simulink model "rolling_contact_36_example"  (R2026b)
settings: Solver=VariableStepAuto  StopTime=5
undefined symbols (not defined in the file): f_rr, k_gx, k_gy, k_x, m_wheel, miu_p, miu_s, mu_slide, mu_stick, omega_rr_eps, r_wheel, sgn, v_gx_max, v_gy_max, vLimit, X, Y, Z
libraries: nesl_utility x225, sm_lib x156, simulink x146, simulink_extras x36
(part 9 of 11)

== system rolling_contact_36_example/36-Point Sliding Contact Model/Body Contact 18/Ground Friction Model/X-Axis Kinetic Friction Model ==
  note: Sliding Limit Detector
  note: Footpoint Determiner
  note: Kinetic Friction Model
  pos [m] : Inport
  vel [m/s] : Inport  Port=2
  F_Normal [N] : Inport  Port=3
  Enable : EnablePort  StatesWhenEnabling=reset  ZeroCross=off
  Abs : Abs  SaturateOnIntegerOverflow=off
  Constant : Constant  Value=vLimit
  FixPt Relational Operator : RelationalOperator  Operator=>  OutDataTypeStr=boolean  ZeroCross=off  InputSameDT=off
  Memory : Memory
  Negative : simulink/Logic and Bit Operations/Compare To Zero  relop=<  OutDataTypeStr=boolean
  Product : Product  RndMeth=Zero
  Sign1 : Signum
  Sum : Sum  Inputs=|+-
  reverse : Gain  Gain=-1
  sliding friction coefficient : Gain  Gain=mu_slide
  posFP [m] : Outport  InitialOutput=0
      settings: AttributesFormatString=initial = '%<InitialOutput>'\nwhen disabled = '%<OutputWhenDisabled>'
  Stiction! : Outport  Port=2  OutputWhenDisabled=reset  InitialOutput=0
      settings: AttributesFormatString=initial = '%<InitialOutput>'\nwhen disabled = '%<OutputWhenDisabled>'
  F_Slide [N] : Outport  Port=3  OutputWhenDisabled=reset  InitialOutput=0
      settings: AttributesFormatString=initial = '%<InitialOutput>'\nwhen disabled = '%<OutputWhenDisabled>'
  wires:
  Constant/1 -> Sum/2
  Sum/1 -> Negative/1
  Abs/1 -> Sum/1
  Negative/1 -> Memory/1, FixPt Relational Operator/1
  Memory/1 -> FixPt Relational Operator/2
  FixPt Relational Operator/1 -> Stiction!/1
  Sign1/1 -> reverse/1
  sliding friction coefficient/1 -> Product/2
  Product/1 -> F_Slide [N]/1
  pos [m]/1 -> posFP [m]/1
  vel [m/s]/1 -> Abs/1, Sign1/1
  F_Normal [N]/1 -> sliding friction coefficient/1
  reverse/1 -> Product/1

== system rolling_contact_36_example/36-Point Sliding Contact Model/Body Contact 18/Ground Friction Model/X-Axis Static Friction Model ==
  note: Static Friction Model
  note: Stiction Limit Detector
  note: Zero multiplication prevents
      | horizontal friction model from
      | oscillating between static and kinetic
      | friction when the vertical force is zero but
      | the ground level is not yet reached
      | in the upward motion
  F_Normal [N] : Inport
  pos [m] : Inport  Port=2
  vel [m/s] : Inport  Port=3
  posFP [m] : Inport  Port=4
  Enable : EnablePort  StatesWhenEnabling=reset  ZeroCross=off
  Abs : Abs  SaturateOnIntegerOverflow=off
  Abs. : Abs  SaturateOnIntegerOverflow=off
  Check Vertical Friction : Product  RndMeth=Zero
  FixPt Relational Operator : RelationalOperator  Operator=>  OutDataTypeStr=boolean  ZeroCross=off  InputSameDT=off
  Gain3 : Gain  Gain=k_gx
  Gain4 : Gain  Gain=1/v_gx_max
  Memory : Memory
  Mux1 : Mux  Inputs=2
  Positive : simulink/Logic and Bit Operations/Compare To Zero  relop=>  OutDataTypeStr=boolean
  Positive1 : simulink/Logic and Bit Operations/Compare To Zero  relop=>  OutDataTypeStr=boolean
  Sum : Sum  Inputs=-+
  Sum2 : Sum  Inputs=-+|
  X-Axis Stiction Force : Fcn  Expr=-u(1) * (1+sgn(u(1))*u(2))
  stiction limit force : Gain  Gain=mu_stick
  F_Stick [N] : Outport  OutputWhenDisabled=reset  InitialOutput=0
      settings: AttributesFormatString=when disabled: %<OutputWhenDisabled>\ninitial: %<InitialOutput>
  Sliding! : Outport  Port=2  OutputWhenDisabled=reset  InitialOutput=0
      settings: AttributesFormatString=when disabled: %<OutputWhenDisabled>\ninitial: %<InitialOutput>
  wires:
  F_Normal [N]/1 -> stiction limit force/1, Positive1/1
  Sum2/1 -> Gain3/1  "dx"
  pos [m]/1 -> Sum2/2
  posFP [m]/1 -> Sum2/1
  vel [m/s]/1 -> Gain4/1
  Sum/1 -> Positive/1
  Memory/1 -> FixPt Relational Operator/2
  Positive/1 -> FixPt Relational Operator/1, Memory/1
  Abs./1 -> Sum/2
  Mux1/1 -> X-Axis Stiction Force/1
  Gain3/1 -> Mux1/1
  Gain4/1 -> Mux1/2
  FixPt Relational Operator/1 -> Sliding!/1
  Abs/1 -> Sum/1
  stiction limit force/1 -> Abs/1
  X-Axis Stiction Force/1 -> Check Vertical Friction/1
  Positive1/1 -> Check Vertical Friction/2
  Check Vertical Friction/1 -> F_Stick [N]/1, Abs./1

== system rolling_contact_36_example/36-Point Sliding Contact Model/Body Contact 19/Ground Friction Model/Friction Switch ==
  note: Static/Kinetic Friction Switch
  Slide! : Inport
  Stick! : Inport  Port=2
  Memory : Memory
  S-R Flip-Flop : simulink_extras/Flip Flops/S-R Flip-Flop  initial_condition=1
  Terminator : Terminator
  Stiction : Outport
  wires:
  S-R Flip-Flop/1 -> Memory/1
  S-R Flip-Flop/2 -> Terminator/1
  Stick!/1 -> S-R Flip-Flop/1
  Slide!/1 -> S-R Flip-Flop/2
  Memory/1 -> Stiction/1

== system rolling_contact_36_example/36-Point Sliding Contact Model/Body Contact 19/Ground Friction Model/X-Axis Kinetic Friction Model ==
  note: Kinetic Friction Model
  note: Footpoint Determiner
  note: Sliding Limit Detector
  pos [m] : Inport
  vel [m/s] : Inport  Port=2
  F_Normal [N] : Inport  Port=3
  Enable : EnablePort  StatesWhenEnabling=reset  ZeroCross=off
  Abs : Abs  SaturateOnIntegerOverflow=off
  Constant : Constant  Value=vLimit
  FixPt Relational Operator : RelationalOperator  Operator=>  OutDataTypeStr=boolean  ZeroCross=off  InputSameDT=off
  Memory : Memory
  Negative : simulink/Logic and Bit Operations/Compare To Zero  relop=<  OutDataTypeStr=boolean
  Product : Product  RndMeth=Zero
  Sign1 : Signum
  Sum : Sum  Inputs=|+-
  reverse : Gain  Gain=-1
  sliding friction coefficient : Gain  Gain=mu_slide
  posFP [m] : Outport  InitialOutput=0
      settings: AttributesFormatString=initial = '%<InitialOutput>'\nwhen disabled = '%<OutputWhenDisabled>'
  Stiction! : Outport  Port=2  OutputWhenDisabled=reset  InitialOutput=0
      settings: AttributesFormatString=initial = '%<InitialOutput>'\nwhen disabled = '%<OutputWhenDisabled>'
  F_Slide [N] : Outport  Port=3  OutputWhenDisabled=reset  InitialOutput=0
      settings: AttributesFormatString=initial = '%<InitialOutput>'\nwhen disabled = '%<OutputWhenDisabled>'
  wires:
  reverse/1 -> Product/1
  F_Normal [N]/1 -> sliding friction coefficient/1
  vel [m/s]/1 -> Sign1/1, Abs/1
  pos [m]/1 -> posFP [m]/1
  Product/1 -> F_Slide [N]/1
  sliding friction coefficient/1 -> Product/2
  Sign1/1 -> reverse/1
  FixPt Relational Operator/1 -> Stiction!/1
  Memory/1 -> FixPt Relational Operator/2
  Negative/1 -> FixPt Relational Operator/1, Memory/1
  Abs/1 -> Sum/1
  Sum/1 -> Negative/1
  Constant/1 -> Sum/2

== system rolling_contact_36_example/36-Point Sliding Contact Model/Body Contact 19/Ground Friction Model/X-Axis Static Friction Model ==
  note: Zero multiplication prevents
      | horizontal friction model from
      | oscillating between static and kinetic
      | friction when the vertical force is zero but
      | the ground level is not yet reached
      | in the upward motion
  note: Stiction Limit Detector
  note: Static Friction Model
  F_Normal [N] : Inport
  pos [m] : Inport  Port=2
  vel [m/s] : Inport  Port=3
  posFP [m] : Inport  Port=4
  Enable : EnablePort  StatesWhenEnabling=reset  ZeroCross=off
  Abs : Abs  SaturateOnIntegerOverflow=off
  Abs. : Abs  SaturateOnIntegerOverflow=off
  Check Vertical Friction : Product  RndMeth=Zero
  FixPt Relational Operator : RelationalOperator  Operator=>  OutDataTypeStr=boolean  ZeroCross=off  InputSameDT=off
  Gain3 : Gain  Gain=k_gx
  Gain4 : Gain  Gain=1/v_gx_max
  Memory : Memory
  Mux1 : Mux  Inputs=2
  Positive : simulink/Logic and Bit Operations/Compare To Zero  relop=>  OutDataTypeStr=boolean
  Positive1 : simulink/Logic and Bit Operations/Compare To Zero  relop=>  OutDataTypeStr=boolean
  Sum : Sum  Inputs=-+
  Sum2 : Sum  Inputs=-+|
  X-Axis Stiction Force : Fcn  Expr=-u(1) * (1+sgn(u(1))*u(2))
  stiction limit force : Gain  Gain=mu_stick
  F_Stick [N] : Outport  OutputWhenDisabled=reset  InitialOutput=0
      settings: AttributesFormatString=when disabled: %<OutputWhenDisabled>\ninitial: %<InitialOutput>
  Sliding! : Outport  Port=2  OutputWhenDisabled=reset  InitialOutput=0
      settings: AttributesFormatString=when disabled: %<OutputWhenDisabled>\ninitial: %<InitialOutput>
  wires:
  Check Vertical Friction/1 -> Abs./1, F_Stick [N]/1
  Positive1/1 -> Check Vertical Friction/2
  X-Axis Stiction Force/1 -> Check Vertical Friction/1
  stiction limit force/1 -> Abs/1
  Abs/1 -> Sum/1
  FixPt Relational Operator/1 -> Sliding!/1
  Gain4/1 -> Mux1/2
  Gain3/1 -> Mux1/1
  Mux1/1 -> X-Axis Stiction Force/1
  Abs./1 -> Sum/2
  Positive/1 -> Memory/1, FixPt Relational Operator/1
  Memory/1 -> FixPt Relational Operator/2
  Sum/1 -> Positive/1
  vel [m/s]/1 -> Gain4/1
  posFP [m]/1 -> Sum2/1
  pos [m]/1 -> Sum2/2
  Sum2/1 -> Gain3/1  "dx"
  F_Normal [N]/1 -> Positive1/1, stiction limit force/1

== system rolling_contact_36_example/36-Point Sliding Contact Model/Body Contact 2/Ground Friction Model/Friction Switch ==
  note: Static/Kinetic Friction Switch
  Slide! : Inport
  Stick! : Inport  Port=2
  Memory : Memory
  S-R Flip-Flop : simulink_extras/Flip Flops/S-R Flip-Flop  initial_condition=1
  Terminator : Terminator
  Stiction : Outport
  wires:
  Memory/1 -> Stiction/1
  Slide!/1 -> S-R Flip-Flop/2
  Stick!/1 -> S-R Flip-Flop/1
  S-R Flip-Flop/2 -> Terminator/1
  S-R Flip-Flop/1 -> Memory/1

== system rolling_contact_36_example/36-Point Sliding Contact Model/Body Contact 2/Ground Friction Model/X-Axis Kinetic Friction Model ==
  note: Sliding Limit Detector
  note: Footpoint Determiner
  note: Kinetic Friction Model
  pos [m] : Inport
  vel [m/s] : Inport  Port=2
  F_Normal [N] : Inport  Port=3
  Enable : EnablePort  StatesWhenEnabling=reset  ZeroCross=off
  Abs : Abs  SaturateOnIntegerOverflow=off
  Constant : Constant  Value=vLimit
  FixPt Relational Operator : RelationalOperator  Operator=>  OutDataTypeStr=boolean  ZeroCross=off  InputSameDT=off
  Memory : Memory
  Negative : simulink/Logic and Bit Operations/Compare To Zero  relop=<  OutDataTypeStr=boolean
  Product : Product  RndMeth=Zero
  Sign1 : Signum
  Sum : Sum  Inputs=|+-
  reverse : Gain  Gain=-1
  sliding friction coefficient : Gain  Gain=mu_slide
  posFP [m] : Outport  InitialOutput=0
      settings: AttributesFormatString=initial = '%<InitialOutput>'\nwhen disabled = '%<OutputWhenDisabled>'
  Stiction! : Outport  Port=2  OutputWhenDisabled=reset  InitialOutput=0
      settings: AttributesFormatString=initial = '%<InitialOutput>'\nwhen disabled = '%<OutputWhenDisabled>'
  F_Slide [N] : Outport  Port=3  OutputWhenDisabled=reset  InitialOutput=0
      settings: AttributesFormatString=initial = '%<InitialOutput>'\nwhen disabled = '%<OutputWhenDisabled>'
  wires:
  Constant/1 -> Sum/2
  Sum/1 -> Negative/1
  Abs/1 -> Sum/1
  Negative/1 -> Memory/1, FixPt Relational Operator/1
  Memory/1 -> FixPt Relational Operator/2
  FixPt Relational Operator/1 -> Stiction!/1
  Sign1/1 -> reverse/1
  sliding friction coefficient/1 -> Product/2
  Product/1 -> F_Slide [N]/1
  pos [m]/1 -> posFP [m]/1
  vel [m/s]/1 -> Abs/1, Sign1/1
  F_Normal [N]/1 -> sliding friction coefficient/1
  reverse/1 -> Product/1

== system rolling_contact_36_example/36-Point Sliding Contact Model/Body Contact 2/Ground Friction Model/X-Axis Static Friction Model ==
  note: Static Friction Model
  note: Stiction Limit Detector
  note: Zero multiplication prevents
      | horizontal friction model from
      | oscillating between static and kinetic
      | friction when the vertical force is zero but
      | the ground level is not yet reached
      | in the upward motion
  F_Normal [N] : Inport
  pos [m] : Inport  Port=2
  vel [m/s] : Inport  Port=3
  posFP [m] : Inport  Port=4
  Enable : EnablePort  StatesWhenEnabling=reset  ZeroCross=off
  Abs : Abs  SaturateOnIntegerOverflow=off
  Abs. : Abs  SaturateOnIntegerOverflow=off
  Check Vertical Friction : Product  RndMeth=Zero
  FixPt Relational Operator : RelationalOperator  Operator=>  OutDataTypeStr=boolean  ZeroCross=off  InputSameDT=off
  Gain3 : Gain  Gain=k_gx
  Gain4 : Gain  Gain=1/v_gx_max
  Memory : Memory
  Mux1 : Mux  Inputs=2
  Positive : simulink/Logic and Bit Operations/Compare To Zero  relop=>  OutDataTypeStr=boolean
  Positive1 : simulink/Logic and Bit Operations/Compare To Zero  relop=>  OutDataTypeStr=boolean
  Sum : Sum  Inputs=-+
  Sum2 : Sum  Inputs=-+|
  X-Axis Stiction Force : Fcn  Expr=-u(1) * (1+sgn(u(1))*u(2))
  stiction limit force : Gain  Gain=mu_stick
  F_Stick [N] : Outport  OutputWhenDisabled=reset  InitialOutput=0
      settings: AttributesFormatString=when disabled: %<OutputWhenDisabled>\ninitial: %<InitialOutput>
  Sliding! : Outport  Port=2  OutputWhenDisabled=reset  InitialOutput=0
      settings: AttributesFormatString=when disabled: %<OutputWhenDisabled>\ninitial: %<InitialOutput>
  wires:
  F_Normal [N]/1 -> stiction limit force/1, Positive1/1
  Sum2/1 -> Gain3/1  "dx"
  pos [m]/1 -> Sum2/2
  posFP [m]/1 -> Sum2/1
  vel [m/s]/1 -> Gain4/1
  Sum/1 -> Positive/1
  Memory/1 -> FixPt Relational Operator/2
  Positive/1 -> FixPt Relational Operator/1, Memory/1
  Abs./1 -> Sum/2
  Mux1/1 -> X-Axis Stiction Force/1
  Gain3/1 -> Mux1/1
  Gain4/1 -> Mux1/2
  FixPt Relational Operator/1 -> Sliding!/1
  Abs/1 -> Sum/1
  stiction limit force/1 -> Abs/1
  X-Axis Stiction Force/1 -> Check Vertical Friction/1
  Positive1/1 -> Check Vertical Friction/2
  Check Vertical Friction/1 -> F_Stick [N]/1, Abs./1

== system rolling_contact_36_example/36-Point Sliding Contact Model/Body Contact 20/Ground Friction Model/Friction Switch ==
  note: Static/Kinetic Friction Switch
  Slide! : Inport
  Stick! : Inport  Port=2
  Memory : Memory
  S-R Flip-Flop : simulink_extras/Flip Flops/S-R Flip-Flop  initial_condition=1
  Terminator : Terminator
  Stiction : Outport
  wires:
  Memory/1 -> Stiction/1
  Slide!/1 -> S-R Flip-Flop/2
  Stick!/1 -> S-R Flip-Flop/1
  S-R Flip-Flop/2 -> Terminator/1
  S-R Flip-Flop/1 -> Memory/1

== system rolling_contact_36_example/36-Point Sliding Contact Model/Body Contact 20/Ground Friction Model/X-Axis Kinetic Friction Model ==
  note: Sliding Limit Detector
  note: Footpoint Determiner
  note: Kinetic Friction Model
  pos [m] : Inport
  vel [m/s] : Inport  Port=2
  F_Normal [N] : Inport  Port=3
  Enable : EnablePort  StatesWhenEnabling=reset  ZeroCross=off
  Abs : Abs  SaturateOnIntegerOverflow=off
  Constant : Constant  Value=vLimit
  FixPt Relational Operator : RelationalOperator  Operator=>  OutDataTypeStr=boolean  ZeroCross=off  InputSameDT=off
  Memory : Memory
  Negative : simulink/Logic and Bit Operations/Compare To Zero  relop=<  OutDataTypeStr=boolean
  Product : Product  RndMeth=Zero
  Sign1 : Signum
  Sum : Sum  Inputs=|+-
  reverse : Gain  Gain=-1
  sliding friction coefficient : Gain  Gain=mu_slide
  posFP [m] : Outport  InitialOutput=0
      settings: AttributesFormatString=initial = '%<InitialOutput>'\nwhen disabled = '%<OutputWhenDisabled>'
  Stiction! : Outport  Port=2  OutputWhenDisabled=reset  InitialOutput=0
      settings: AttributesFormatString=initial = '%<InitialOutput>'\nwhen disabled = '%<OutputWhenDisabled>'
  F_Slide [N] : Outport  Port=3  OutputWhenDisabled=reset  InitialOutput=0
      settings: AttributesFormatString=initial = '%<InitialOutput>'\nwhen disabled = '%<OutputWhenDisabled>'
  wires:
  Constant/1 -> Sum/2
  Sum/1 -> Negative/1
  Abs/1 -> Sum/1
  Negative/1 -> Memory/1, FixPt Relational Operator/1
  Memory/1 -> FixPt Relational Operator/2
  FixPt Relational Operator/1 -> Stiction!/1
  Sign1/1 -> reverse/1
  sliding friction coefficient/1 -> Product/2
  Product/1 -> F_Slide [N]/1
  pos [m]/1 -> posFP [m]/1
  vel [m/s]/1 -> Abs/1, Sign1/1
  F_Normal [N]/1 -> sliding friction coefficient/1
  reverse/1 -> Product/1

== system rolling_contact_36_example/36-Point Sliding Contact Model/Body Contact 20/Ground Friction Model/X-Axis Static Friction Model ==
  note: Static Friction Model
  note: Stiction Limit Detector
  note: Zero multiplication prevents
      | horizontal friction model from
      | oscillating between static and kinetic
      | friction when the vertical force is zero but
      | the ground level is not yet reached
      | in the upward motion
  F_Normal [N] : Inport
  pos [m] : Inport  Port=2
  vel [m/s] : Inport  Port=3
  posFP [m] : Inport  Port=4
  Enable : EnablePort  StatesWhenEnabling=reset  ZeroCross=off
  Abs : Abs  SaturateOnIntegerOverflow=off
  Abs. : Abs  SaturateOnIntegerOverflow=off
  Check Vertical Friction : Product  RndMeth=Zero
  FixPt Relational Operator : RelationalOperator  Operator=>  OutDataTypeStr=boolean  ZeroCross=off  InputSameDT=off
  Gain3 : Gain  Gain=k_gx
  Gain4 : Gain  Gain=1/v_gx_max
  Memory : Memory
  Mux1 : Mux  Inputs=2
  Positive : simulink/Logic and Bit Operations/Compare To Zero  relop=>  OutDataTypeStr=boolean
  Positive1 : simulink/Logic and Bit Operations/Compare To Zero  relop=>  OutDataTypeStr=boolean
  Sum : Sum  Inputs=-+
  Sum2 : Sum  Inputs=-+|
  X-Axis Stiction Force : Fcn  Expr=-u(1) * (1+sgn(u(1))*u(2))
  stiction limit force : Gain  Gain=mu_stick
  F_Stick [N] : Outport  OutputWhenDisabled=reset  InitialOutput=0
      settings: AttributesFormatString=when disabled: %<OutputWhenDisabled>\ninitial: %<InitialOutput>
  Sliding! : Outport  Port=2  OutputWhenDisabled=reset  InitialOutput=0
      settings: AttributesFormatString=when disabled: %<OutputWhenDisabled>\ninitial: %<InitialOutput>
  wires:
  F_Normal [N]/1 -> stiction limit force/1, Positive1/1
  Sum2/1 -> Gain3/1  "dx"
  pos [m]/1 -> Sum2/2
  posFP [m]/1 -> Sum2/1
  vel [m/s]/1 -> Gain4/1
  Sum/1 -> Positive/1
  Memory/1 -> FixPt Relational Operator/2
  Positive/1 -> FixPt Relational Operator/1, Memory/1
  Abs./1 -> Sum/2
  Mux1/1 -> X-Axis Stiction Force/1
  Gain3/1 -> Mux1/1
  Gain4/1 -> Mux1/2
  FixPt Relational Operator/1 -> Sliding!/1
  Abs/1 -> Sum/1
  stiction limit force/1 -> Abs/1
  X-Axis Stiction Force/1 -> Check Vertical Friction/1
  Positive1/1 -> Check Vertical Friction/2
  Check Vertical Friction/1 -> F_Stick [N]/1, Abs./1

== system rolling_contact_36_example/36-Point Sliding Contact Model/Body Contact 21/Ground Friction Model/Friction Switch ==
  note: Static/Kinetic Friction Switch
  Slide! : Inport
  Stick! : Inport  Port=2
  Memory : Memory
  S-R Flip-Flop : simulink_extras/Flip Flops/S-R Flip-Flop  initial_condition=1
  Terminator : Terminator
  Stiction : Outport
  wires:
  S-R Flip-Flop/1 -> Memory/1
  S-R Flip-Flop/2 -> Terminator/1
  Stick!/1 -> S-R Flip-Flop/1
  Slide!/1 -> S-R Flip-Flop/2
  Memory/1 -> Stiction/1

== system rolling_contact_36_example/36-Point Sliding Contact Model/Body Contact 21/Ground Friction Model/X-Axis Kinetic Friction Model ==
  note: Kinetic Friction Model
  note: Footpoint Determiner
  note: Sliding Limit Detector
  pos [m] : Inport
  vel [m/s] : Inport  Port=2
  F_Normal [N] : Inport  Port=3
  Enable : EnablePort  StatesWhenEnabling=reset  ZeroCross=off
  Abs : Abs  SaturateOnIntegerOverflow=off
  Constant : Constant  Value=vLimit
  FixPt Relational Operator : RelationalOperator  Operator=>  OutDataTypeStr=boolean  ZeroCross=off  InputSameDT=off
  Memory : Memory
  Negative : simulink/Logic and Bit Operations/Compare To Zero  relop=<  OutDataTypeStr=boolean
  Product : Product  RndMeth=Zero
  Sign1 : Signum
  Sum : Sum  Inputs=|+-
  reverse : Gain  Gain=-1
  sliding friction coefficient : Gain  Gain=mu_slide
  posFP [m] : Outport  InitialOutput=0
      settings: AttributesFormatString=initial = '%<InitialOutput>'\nwhen disabled = '%<OutputWhenDisabled>'
  Stiction! : Outport  Port=2  OutputWhenDisabled=reset  InitialOutput=0
      settings: AttributesFormatString=initial = '%<InitialOutput>'\nwhen disabled = '%<OutputWhenDisabled>'
  F_Slide [N] : Outport  Port=3  OutputWhenDisabled=reset  InitialOutput=0
      settings: AttributesFormatString=initial = '%<InitialOutput>'\nwhen disabled = '%<OutputWhenDisabled>'
  wires:
  reverse/1 -> Product/1
  F_Normal [N]/1 -> sliding friction coefficient/1
  vel [m/s]/1 -> Sign1/1, Abs/1
  pos [m]/1 -> posFP [m]/1
  Product/1 -> F_Slide [N]/1
  sliding friction coefficient/1 -> Product/2
  Sign1/1 -> reverse/1
  FixPt Relational Operator/1 -> Stiction!/1
  Memory/1 -> FixPt Relational Operator/2
  Negative/1 -> FixPt Relational Operator/1, Memory/1
  Abs/1 -> Sum/1
  Sum/1 -> Negative/1
  Constant/1 -> Sum/2

== system rolling_contact_36_example/36-Point Sliding Contact Model/Body Contact 21/Ground Friction Model/X-Axis Static Friction Model ==
  note: Zero multiplication prevents
      | horizontal friction model from
      | oscillating between static and kinetic
      | friction when the vertical force is zero but
      | the ground level is not yet reached
      | in the upward motion
  note: Stiction Limit Detector
  note: Static Friction Model
  F_Normal [N] : Inport
  pos [m] : Inport  Port=2
  vel [m/s] : Inport  Port=3
  posFP [m] : Inport  Port=4
  Enable : EnablePort  StatesWhenEnabling=reset  ZeroCross=off
  Abs : Abs  SaturateOnIntegerOverflow=off
  Abs. : Abs  SaturateOnIntegerOverflow=off
  Check Vertical Friction : Product  RndMeth=Zero
  FixPt Relational Operator : RelationalOperator  Operator=>  OutDataTypeStr=boolean  ZeroCross=off  InputSameDT=off
  Gain3 : Gain  Gain=k_gx
  Gain4 : Gain  Gain=1/v_gx_max
  Memory : Memory
  Mux1 : Mux  Inputs=2
  Positive : simulink/Logic and Bit Operations/Compare To Zero  relop=>  OutDataTypeStr=boolean
  Positive1 : simulink/Logic and Bit Operations/Compare To Zero  relop=>  OutDataTypeStr=boolean
  Sum : Sum  Inputs=-+
  Sum2 : Sum  Inputs=-+|
  X-Axis Stiction Force : Fcn  Expr=-u(1) * (1+sgn(u(1))*u(2))
  stiction limit force : Gain  Gain=mu_stick
  F_Stick [N] : Outport  OutputWhenDisabled=reset  InitialOutput=0
      settings: AttributesFormatString=when disabled: %<OutputWhenDisabled>\ninitial: %<InitialOutput>
  Sliding! : Outport  Port=2  OutputWhenDisabled=reset  InitialOutput=0
      settings: AttributesFormatString=when disabled: %<OutputWhenDisabled>\ninitial: %<InitialOutput>
  wires:
  Check Vertical Friction/1 -> Abs./1, F_Stick [N]/1
  Positive1/1 -> Check Vertical Friction/2
  X-Axis Stiction Force/1 -> Check Vertical Friction/1
  stiction limit force/1 -> Abs/1
  Abs/1 -> Sum/1
  FixPt Relational Operator/1 -> Sliding!/1
  Gain4/1 -> Mux1/2
  Gain3/1 -> Mux1/1
  Mux1/1 -> X-Axis Stiction Force/1
  Abs./1 -> Sum/2
  Positive/1 -> Memory/1, FixPt Relational Operator/1
  Memory/1 -> FixPt Relational Operator/2
  Sum/1 -> Positive/1
  vel [m/s]/1 -> Gain4/1
  posFP [m]/1 -> Sum2/1
  pos [m]/1 -> Sum2/2
  Sum2/1 -> Gain3/1  "dx"
  F_Normal [N]/1 -> Positive1/1, stiction limit force/1

== system rolling_contact_36_example/36-Point Sliding Contact Model/Body Contact 22/Ground Friction Model/Friction Switch ==
  note: Static/Kinetic Friction Switch
  Slide! : Inport
  Stick! : Inport  Port=2
  Memory : Memory
  S-R Flip-Flop : simulink_extras/Flip Flops/S-R Flip-Flop  initial_condition=1
  Terminator : Terminator
  Stiction : Outport
  wires:
  Memory/1 -> Stiction/1
  Slide!/1 -> S-R Flip-Flop/2
  Stick!/1 -> S-R Flip-Flop/1
  S-R Flip-Flop/2 -> Terminator/1
  S-R Flip-Flop/1 -> Memory/1

== system rolling_contact_36_example/36-Point Sliding Contact Model/Body Contact 22/Ground Friction Model/X-Axis Kinetic Friction Model ==
  note: Sliding Limit Detector
  note: Footpoint Determiner
  note: Kinetic Friction Model
  pos [m] : Inport
  vel [m/s] : Inport  Port=2
  F_Normal [N] : Inport  Port=3
  Enable : EnablePort  StatesWhenEnabling=reset  ZeroCross=off
  Abs : Abs  SaturateOnIntegerOverflow=off
  Constant : Constant  Value=vLimit
  FixPt Relational Operator : RelationalOperator  Operator=>  OutDataTypeStr=boolean  ZeroCross=off  InputSameDT=off
  Memory : Memory
  Negative : simulink/Logic and Bit Operations/Compare To Zero  relop=<  OutDataTypeStr=boolean
  Product : Product  RndMeth=Zero
  Sign1 : Signum
  Sum : Sum  Inputs=|+-
  reverse : Gain  Gain=-1
  sliding friction coefficient : Gain  Gain=mu_slide
  posFP [m] : Outport  InitialOutput=0
      settings: AttributesFormatString=initial = '%<InitialOutput>'\nwhen disabled = '%<OutputWhenDisabled>'
  Stiction! : Outport  Port=2  OutputWhenDisabled=reset  InitialOutput=0
      settings: AttributesFormatString=initial = '%<InitialOutput>'\nwhen disabled = '%<OutputWhenDisabled>'
  F_Slide [N] : Outport  Port=3  OutputWhenDisabled=reset  InitialOutput=0
      settings: AttributesFormatString=initial = '%<InitialOutput>'\nwhen disabled = '%<OutputWhenDisabled>'
  wires:
  Constant/1 -> Sum/2
  Sum/1 -> Negative/1
  Abs/1 -> Sum/1
  Negative/1 -> Memory/1, FixPt Relational Operator/1
  Memory/1 -> FixPt Relational Operator/2
  FixPt Relational Operator/1 -> Stiction!/1
  Sign1/1 -> reverse/1
  sliding friction coefficient/1 -> Product/2
  Product/1 -> F_Slide [N]/1
  pos [m]/1 -> posFP [m]/1
  vel [m/s]/1 -> Abs/1, Sign1/1
  F_Normal [N]/1 -> sliding friction coefficient/1
  reverse/1 -> Product/1

== system rolling_contact_36_example/36-Point Sliding Contact Model/Body Contact 22/Ground Friction Model/X-Axis Static Friction Model ==
  note: Static Friction Model
  note: Stiction Limit Detector
  note: Zero multiplication prevents
      | horizontal friction model from
      | oscillating between static and kinetic
      | friction when the vertical force is zero but
      | the ground level is not yet reached
      | in the upward motion
  F_Normal [N] : Inport
  pos [m] : Inport  Port=2
  vel [m/s] : Inport  Port=3
  posFP [m] : Inport  Port=4
  Enable : EnablePort  StatesWhenEnabling=reset  ZeroCross=off
  Abs : Abs  SaturateOnIntegerOverflow=off
  Abs. : Abs  SaturateOnIntegerOverflow=off
  Check Vertical Friction : Product  RndMeth=Zero
  FixPt Relational Operator : RelationalOperator  Operator=>  OutDataTypeStr=boolean  ZeroCross=off  InputSameDT=off
  Gain3 : Gain  Gain=k_gx
  Gain4 : Gain  Gain=1/v_gx_max
  Memory : Memory
  Mux1 : Mux  Inputs=2
  Positive : simulink/Logic and Bit Operations/Compare To Zero  relop=>  OutDataTypeStr=boolean
  Positive1 : simulink/Logic and Bit Operations/Compare To Zero  relop=>  OutDataTypeStr=boolean
  Sum : Sum  Inputs=-+
  Sum2 : Sum  Inputs=-+|
  X-Axis Stiction Force : Fcn  Expr=-u(1) * (1+sgn(u(1))*u(2))
  stiction limit force : Gain  Gain=mu_stick
  F_Stick [N] : Outport  OutputWhenDisabled=reset  InitialOutput=0
      settings: AttributesFormatString=when disabled: %<OutputWhenDisabled>\ninitial: %<InitialOutput>
  Sliding! : Outport  Port=2  OutputWhenDisabled=reset  InitialOutput=0
      settings: AttributesFormatString=when disabled: %<OutputWhenDisabled>\ninitial: %<InitialOutput>
  wires:
  F_Normal [N]/1 -> stiction limit force/1, Positive1/1
  Sum2/1 -> Gain3/1  "dx"
  pos [m]/1 -> Sum2/2
  posFP [m]/1 -> Sum2/1
  vel [m/s]/1 -> Gain4/1
  Sum/1 -> Positive/1
  Memory/1 -> FixPt Relational Operator/2
  Positive/1 -> FixPt Relational Operator/1, Memory/1
  Abs./1 -> Sum/2
  Mux1/1 -> X-Axis Stiction Force/1
  Gain3/1 -> Mux1/1
  Gain4/1 -> Mux1/2
  FixPt Relational Operator/1 -> Sliding!/1
  Abs/1 -> Sum/1
  stiction limit force/1 -> Abs/1
  X-Axis Stiction Force/1 -> Check Vertical Friction/1
  Positive1/1 -> Check Vertical Friction/2
  Check Vertical Friction/1 -> F_Stick [N]/1, Abs./1

== system rolling_contact_36_example/36-Point Sliding Contact Model/Body Contact 23/Ground Friction Model/Friction Switch ==
  note: Static/Kinetic Friction Switch
  Slide! : Inport
  Stick! : Inport  Port=2
  Memory : Memory
  S-R Flip-Flop : simulink_extras/Flip Flops/S-R Flip-Flop  initial_condition=1
  Terminator : Terminator
  Stiction : Outport
  wires:
  S-R Flip-Flop/1 -> Memory/1
  S-R Flip-Flop/2 -> Terminator/1
  Stick!/1 -> S-R Flip-Flop/1
  Slide!/1 -> S-R Flip-Flop/2
  Memory/1 -> Stiction/1

== system rolling_contact_36_example/36-Point Sliding Contact Model/Body Contact 23/Ground Friction Model/X-Axis Kinetic Friction Model ==
  note: Kinetic Friction Model
  note: Footpoint Determiner
  note: Sliding Limit Detector
  pos [m] : Inport
  vel [m/s] : Inport  Port=2
  F_Normal [N] : Inport  Port=3
  Enable : EnablePort  StatesWhenEnabling=reset  ZeroCross=off
  Abs : Abs  SaturateOnIntegerOverflow=off
  Constant : Constant  Value=vLimit
  FixPt Relational Operator : RelationalOperator  Operator=>  OutDataTypeStr=boolean  ZeroCross=off  InputSameDT=off
  Memory : Memory
  Negative : simulink/Logic and Bit Operations/Compare To Zero  relop=<  OutDataTypeStr=boolean
  Product : Product  RndMeth=Zero
  Sign1 : Signum
  Sum : Sum  Inputs=|+-
  reverse : Gain  Gain=-1
  sliding friction coefficient : Gain  Gain=mu_slide
  posFP [m] : Outport  InitialOutput=0
      settings: AttributesFormatString=initial = '%<InitialOutput>'\nwhen disabled = '%<OutputWhenDisabled>'
  Stiction! : Outport  Port=2  OutputWhenDisabled=reset  InitialOutput=0
      settings: AttributesFormatString=initial = '%<InitialOutput>'\nwhen disabled = '%<OutputWhenDisabled>'
  F_Slide [N] : Outport  Port=3  OutputWhenDisabled=reset  InitialOutput=0
      settings: AttributesFormatString=initial = '%<InitialOutput>'\nwhen disabled = '%<OutputWhenDisabled>'
  wires:
  reverse/1 -> Product/1
  F_Normal [N]/1 -> sliding friction coefficient/1
  vel [m/s]/1 -> Sign1/1, Abs/1
  pos [m]/1 -> posFP [m]/1
  Product/1 -> F_Slide [N]/1
  sliding friction coefficient/1 -> Product/2
  Sign1/1 -> reverse/1
  FixPt Relational Operator/1 -> Stiction!/1
  Memory/1 -> FixPt Relational Operator/2
  Negative/1 -> FixPt Relational Operator/1, Memory/1
  Abs/1 -> Sum/1
  Sum/1 -> Negative/1
  Constant/1 -> Sum/2

== system rolling_contact_36_example/36-Point Sliding Contact Model/Body Contact 23/Ground Friction Model/X-Axis Static Friction Model ==
  note: Zero multiplication prevents
      | horizontal friction model from
      | oscillating between static and kinetic
      | friction when the vertical force is zero but
      | the ground level is not yet reached
      | in the upward motion
  note: Stiction Limit Detector
  note: Static Friction Model
  F_Normal [N] : Inport
  pos [m] : Inport  Port=2
  vel [m/s] : Inport  Port=3
  posFP [m] : Inport  Port=4
  Enable : EnablePort  StatesWhenEnabling=reset  ZeroCross=off
  Abs : Abs  SaturateOnIntegerOverflow=off
  Abs. : Abs  SaturateOnIntegerOverflow=off
  Check Vertical Friction : Product  RndMeth=Zero
  FixPt Relational Operator : RelationalOperator  Operator=>  OutDataTypeStr=boolean  ZeroCross=off  InputSameDT=off
  Gain3 : Gain  Gain=k_gx
  Gain4 : Gain  Gain=1/v_gx_max
  Memory : Memory
  Mux1 : Mux  Inputs=2
  Positive : simulink/Logic and Bit Operations/Compare To Zero  relop=>  OutDataTypeStr=boolean
  Positive1 : simulink/Logic and Bit Operations/Compare To Zero  relop=>  OutDataTypeStr=boolean
  Sum : Sum  Inputs=-+
  Sum2 : Sum  Inputs=-+|
  X-Axis Stiction Force : Fcn  Expr=-u(1) * (1+sgn(u(1))*u(2))
  stiction limit force : Gain  Gain=mu_stick
  F_Stick [N] : Outport  OutputWhenDisabled=reset  InitialOutput=0
      settings: AttributesFormatString=when disabled: %<OutputWhenDisabled>\ninitial: %<InitialOutput>
  Sliding! : Outport  Port=2  OutputWhenDisabled=reset  InitialOutput=0
      settings: AttributesFormatString=when disabled: %<OutputWhenDisabled>\ninitial: %<InitialOutput>
  wires:
  Check Vertical Friction/1 -> Abs./1, F_Stick [N]/1
  Positive1/1 -> Check Vertical Friction/2
  X-Axis Stiction Force/1 -> Check Vertical Friction/1
  stiction limit force/1 -> Abs/1
  Abs/1 -> Sum/1
  FixPt Relational Operator/1 -> Sliding!/1
  Gain4/1 -> Mux1/2
  Gain3/1 -> Mux1/1
  Mux1/1 -> X-Axis Stiction Force/1
  Abs./1 -> Sum/2
  Positive/1 -> Memory/1, FixPt Relational Operator/1
  Memory/1 -> FixPt Relational Operator/2
  Sum/1 -> Positive/1
  vel [m/s]/1 -> Gain4/1
  posFP [m]/1 -> Sum2/1
  pos [m]/1 -> Sum2/2
  Sum2/1 -> Gain3/1  "dx"
  F_Normal [N]/1 -> Positive1/1, stiction limit force/1

== system rolling_contact_36_example/36-Point Sliding Contact Model/Body Contact 24/Ground Friction Model/Friction Switch ==
  note: Static/Kinetic Friction Switch
  Slide! : Inport
  Stick! : Inport  Port=2
  Memory : Memory
  S-R Flip-Flop : simulink_extras/Flip Flops/S-R Flip-Flop  initial_condition=1
  Terminator : Terminator
  Stiction : Outport
  wires:
  Memory/1 -> Stiction/1
  Slide!/1 -> S-R Flip-Flop/2
  Stick!/1 -> S-R Flip-Flop/1
  S-R Flip-Flop/2 -> Terminator/1
  S-R Flip-Flop/1 -> Memory/1

== system rolling_contact_36_example/36-Point Sliding Contact Model/Body Contact 24/Ground Friction Model/X-Axis Kinetic Friction Model ==
  note: Sliding Limit Detector
  note: Footpoint Determiner
  note: Kinetic Friction Model
  pos [m] : Inport
  vel [m/s] : Inport  Port=2
  F_Normal [N] : Inport  Port=3
  Enable : EnablePort  StatesWhenEnabling=reset  ZeroCross=off
  Abs : Abs  SaturateOnIntegerOverflow=off
  Constant : Constant  Value=vLimit
  FixPt Relational Operator : RelationalOperator  Operator=>  OutDataTypeStr=boolean  ZeroCross=off  InputSameDT=off
  Memory : Memory
  Negative : simulink/Logic and Bit Operations/Compare To Zero  relop=<  OutDataTypeStr=boolean
  Product : Product  RndMeth=Zero
  Sign1 : Signum
  Sum : Sum  Inputs=|+-
  reverse : Gain  Gain=-1
  sliding friction coefficient : Gain  Gain=mu_slide
  posFP [m] : Outport  InitialOutput=0
      settings: AttributesFormatString=initial = '%<InitialOutput>'\nwhen disabled = '%<OutputWhenDisabled>'
  Stiction! : Outport  Port=2  OutputWhenDisabled=reset  InitialOutput=0
      settings: AttributesFormatString=initial = '%<InitialOutput>'\nwhen disabled = '%<OutputWhenDisabled>'
  F_Slide [N] : Outport  Port=3  OutputWhenDisabled=reset  InitialOutput=0
      settings: AttributesFormatString=initial = '%<InitialOutput>'\nwhen disabled = '%<OutputWhenDisabled>'
  wires:
  Constant/1 -> Sum/2
  Sum/1 -> Negative/1
  Abs/1 -> Sum/1
  Negative/1 -> Memory/1, FixPt Relational Operator/1
  Memory/1 -> FixPt Relational Operator/2
  FixPt Relational Operator/1 -> Stiction!/1
  Sign1/1 -> reverse/1
  sliding friction coefficient/1 -> Product/2
  Product/1 -> F_Slide [N]/1
  pos [m]/1 -> posFP [m]/1
  vel [m/s]/1 -> Abs/1, Sign1/1
  F_Normal [N]/1 -> sliding friction coefficient/1
  reverse/1 -> Product/1

== system rolling_contact_36_example/36-Point Sliding Contact Model/Body Contact 24/Ground Friction Model/X-Axis Static Friction Model ==
  note: Static Friction Model
  note: Stiction Limit Detector
  note: Zero multiplication prevents
      | horizontal friction model from
      | oscillating between static and kinetic
      | friction when the vertical force is zero but
      | the ground level is not yet reached
      | in the upward motion
  F_Normal [N] : Inport
  pos [m] : Inport  Port=2
  vel [m/s] : Inport  Port=3
  posFP [m] : Inport  Port=4
  Enable : EnablePort  StatesWhenEnabling=reset  ZeroCross=off
  Abs : Abs  SaturateOnIntegerOverflow=off
  Abs. : Abs  SaturateOnIntegerOverflow=off
  Check Vertical Friction : Product  RndMeth=Zero
  FixPt Relational Operator : RelationalOperator  Operator=>  OutDataTypeStr=boolean  ZeroCross=off  InputSameDT=off
  Gain3 : Gain  Gain=k_gx
  Gain4 : Gain  Gain=1/v_gx_max
  Memory : Memory
  Mux1 : Mux  Inputs=2
  Positive : simulink/Logic and Bit Operations/Compare To Zero  relop=>  OutDataTypeStr=boolean
  Positive1 : simulink/Logic and Bit Operations/Compare To Zero  relop=>  OutDataTypeStr=boolean
  Sum : Sum  Inputs=-+
  Sum2 : Sum  Inputs=-+|
  X-Axis Stiction Force : Fcn  Expr=-u(1) * (1+sgn(u(1))*u(2))
  stiction limit force : Gain  Gain=mu_stick
  F_Stick [N] : Outport  OutputWhenDisabled=reset  InitialOutput=0
      settings: AttributesFormatString=when disabled: %<OutputWhenDisabled>\ninitial: %<InitialOutput>
  Sliding! : Outport  Port=2  OutputWhenDisabled=reset  InitialOutput=0
      settings: AttributesFormatString=when disabled: %<OutputWhenDisabled>\ninitial: %<InitialOutput>
  wires:
  F_Normal [N]/1 -> stiction limit force/1, Positive1/1
  Sum2/1 -> Gain3/1  "dx"
  pos [m]/1 -> Sum2/2
  posFP [m]/1 -> Sum2/1
  vel [m/s]/1 -> Gain4/1
  Sum/1 -> Positive/1
  Memory/1 -> FixPt Relational Operator/2
  Positive/1 -> FixPt Relational Operator/1, Memory/1
  Abs./1 -> Sum/2
  Mux1/1 -> X-Axis Stiction Force/1
  Gain3/1 -> Mux1/1
  Gain4/1 -> Mux1/2
  FixPt Relational Operator/1 -> Sliding!/1
  Abs/1 -> Sum/1
  stiction limit force/1 -> Abs/1
  X-Axis Stiction Force/1 -> Check Vertical Friction/1
  Positive1/1 -> Check Vertical Friction/2
  Check Vertical Friction/1 -> F_Stick [N]/1, Abs./1

== system rolling_contact_36_example/36-Point Sliding Contact Model/Body Contact 25/Ground Friction Model/Friction Switch ==
  note: Static/Kinetic Friction Switch
  Slide! : Inport
  Stick! : Inport  Port=2
  Memory : Memory
  S-R Flip-Flop : simulink_extras/Flip Flops/S-R Flip-Flop  initial_condition=1
  Terminator : Terminator
  Stiction : Outport
  wires:
  S-R Flip-Flop/1 -> Memory/1
  S-R Flip-Flop/2 -> Terminator/1
  Stick!/1 -> S-R Flip-Flop/1
  Slide!/1 -> S-R Flip-Flop/2
  Memory/1 -> Stiction/1

== system rolling_contact_36_example/36-Point Sliding Contact Model/Body Contact 25/Ground Friction Model/X-Axis Kinetic Friction Model ==
  note: Kinetic Friction Model
  note: Footpoint Determiner
  note: Sliding Limit Detector
  pos [m] : Inport
  vel [m/s] : Inport  Port=2
  F_Normal [N] : Inport  Port=3
  Enable : EnablePort  StatesWhenEnabling=reset  ZeroCross=off
  Abs : Abs  SaturateOnIntegerOverflow=off
  Constant : Constant  Value=vLimit
  FixPt Relational Operator : RelationalOperator  Operator=>  OutDataTypeStr=boolean  ZeroCross=off  InputSameDT=off
  Memory : Memory
  Negative : simulink/Logic and Bit Operations/Compare To Zero  relop=<  OutDataTypeStr=boolean
  Product : Product  RndMeth=Zero
  Sign1 : Signum
  Sum : Sum  Inputs=|+-
  reverse : Gain  Gain=-1
  sliding friction coefficient : Gain  Gain=mu_slide
  posFP [m] : Outport  InitialOutput=0
      settings: AttributesFormatString=initial = '%<InitialOutput>'\nwhen disabled = '%<OutputWhenDisabled>'
  Stiction! : Outport  Port=2  OutputWhenDisabled=reset  InitialOutput=0
      settings: AttributesFormatString=initial = '%<InitialOutput>'\nwhen disabled = '%<OutputWhenDisabled>'
  F_Slide [N] : Outport  Port=3  OutputWhenDisabled=reset  InitialOutput=0
      settings: AttributesFormatString=initial = '%<InitialOutput>'\nwhen disabled = '%<OutputWhenDisabled>'
  wires:
  reverse/1 -> Product/1
  F_Normal [N]/1 -> sliding friction coefficient/1
  vel [m/s]/1 -> Sign1/1, Abs/1
  pos [m]/1 -> posFP [m]/1
  Product/1 -> F_Slide [N]/1
  sliding friction coefficient/1 -> Product/2
  Sign1/1 -> reverse/1
  FixPt Relational Operator/1 -> Stiction!/1
  Memory/1 -> FixPt Relational Operator/2
  Negative/1 -> FixPt Relational Operator/1, Memory/1
  Abs/1 -> Sum/1
  Sum/1 -> Negative/1
  Constant/1 -> Sum/2

== system rolling_contact_36_example/36-Point Sliding Contact Model/Body Contact 25/Ground Friction Model/X-Axis Static Friction Model ==
  note: Zero multiplication prevents
      | horizontal friction model from
      | oscillating between static and kinetic
      | friction when the vertical force is zero but
      | the ground level is not yet reached
      | in the upward motion
  note: Stiction Limit Detector
  note: Static Friction Model
  F_Normal [N] : Inport
  pos [m] : Inport  Port=2
  vel [m/s] : Inport  Port=3
  posFP [m] : Inport  Port=4
  Enable : EnablePort  StatesWhenEnabling=reset  ZeroCross=off
  Abs : Abs  SaturateOnIntegerOverflow=off
  Abs. : Abs  SaturateOnIntegerOverflow=off
  Check Vertical Friction : Product  RndMeth=Zero
  FixPt Relational Operator : RelationalOperator  Operator=>  OutDataTypeStr=boolean  ZeroCross=off  InputSameDT=off
  Gain3 : Gain  Gain=k_gx
  Gain4 : Gain  Gain=1/v_gx_max
  Memory : Memory
  Mux1 : Mux  Inputs=2
  Positive : simulink/Logic and Bit Operations/Compare To Zero  relop=>  OutDataTypeStr=boolean
  Positive1 : simulink/Logic and Bit Operations/Compare To Zero  relop=>  OutDataTypeStr=boolean
  Sum : Sum  Inputs=-+
  Sum2 : Sum  Inputs=-+|
  X-Axis Stiction Force : Fcn  Expr=-u(1) * (1+sgn(u(1))*u(2))
  stiction limit force : Gain  Gain=mu_stick
  F_Stick [N] : Outport  OutputWhenDisabled=reset  InitialOutput=0
      settings: AttributesFormatString=when disabled: %<OutputWhenDisabled>\ninitial: %<InitialOutput>
  Sliding! : Outport  Port=2  OutputWhenDisabled=reset  InitialOutput=0
      settings: AttributesFormatString=when disabled: %<OutputWhenDisabled>\ninitial: %<InitialOutput>
  wires:
  Check Vertical Friction/1 -> Abs./1, F_Stick [N]/1
  Positive1/1 -> Check Vertical Friction/2
  X-Axis Stiction Force/1 -> Check Vertical Friction/1
  stiction limit force/1 -> Abs/1
  Abs/1 -> Sum/1
  FixPt Relational Operator/1 -> Sliding!/1
  Gain4/1 -> Mux1/2
  Gain3/1 -> Mux1/1
  Mux1/1 -> X-Axis Stiction Force/1
  Abs./1 -> Sum/2
  Positive/1 -> Memory/1, FixPt Relational Operator/1
  Memory/1 -> FixPt Relational Operator/2
  Sum/1 -> Positive/1
  vel [m/s]/1 -> Gain4/1
  posFP [m]/1 -> Sum2/1
  pos [m]/1 -> Sum2/2
  Sum2/1 -> Gain3/1  "dx"
  F_Normal [N]/1 -> Positive1/1, stiction limit force/1

== system rolling_contact_36_example/36-Point Sliding Contact Model/Body Contact 26/Ground Friction Model/Friction Switch ==
  note: Static/Kinetic Friction Switch
  Slide! : Inport
  Stick! : Inport  Port=2
  Memory : Memory
  S-R Flip-Flop : simulink_extras/Flip Flops/S-R Flip-Flop  initial_condition=1
  Terminator : Terminator
  Stiction : Outport
  wires:
  Memory/1 -> Stiction/1
  Slide!/1 -> S-R Flip-Flop/2
  Stick!/1 -> S-R Flip-Flop/1
  S-R Flip-Flop/2 -> Terminator/1
  S-R Flip-Flop/1 -> Memory/1

== system rolling_contact_36_example/36-Point Sliding Contact Model/Body Contact 26/Ground Friction Model/X-Axis Kinetic Friction Model ==
  note: Sliding Limit Detector
  note: Footpoint Determiner
  note: Kinetic Friction Model
  pos [m] : Inport
  vel [m/s] : Inport  Port=2
  F_Normal [N] : Inport  Port=3
  Enable : EnablePort  StatesWhenEnabling=reset  ZeroCross=off
  Abs : Abs  SaturateOnIntegerOverflow=off
  Constant : Constant  Value=vLimit
  FixPt Relational Operator : RelationalOperator  Operator=>  OutDataTypeStr=boolean  ZeroCross=off  InputSameDT=off
  Memory : Memory
  Negative : simulink/Logic and Bit Operations/Compare To Zero  relop=<  OutDataTypeStr=boolean
  Product : Product  RndMeth=Zero
  Sign1 : Signum
  Sum : Sum  Inputs=|+-
  reverse : Gain  Gain=-1
  sliding friction coefficient : Gain  Gain=mu_slide
  posFP [m] : Outport  InitialOutput=0
      settings: AttributesFormatString=initial = '%<InitialOutput>'\nwhen disabled = '%<OutputWhenDisabled>'
  Stiction! : Outport  Port=2  OutputWhenDisabled=reset  InitialOutput=0
      settings: AttributesFormatString=initial = '%<InitialOutput>'\nwhen disabled = '%<OutputWhenDisabled>'
  F_Slide [N] : Outport  Port=3  OutputWhenDisabled=reset  InitialOutput=0
      settings: AttributesFormatString=initial = '%<InitialOutput>'\nwhen disabled = '%<OutputWhenDisabled>'
  wires:
  Constant/1 -> Sum/2
  Sum/1 -> Negative/1
  Abs/1 -> Sum/1
  Negative/1 -> Memory/1, FixPt Relational Operator/1
  Memory/1 -> FixPt Relational Operator/2
  FixPt Relational Operator/1 -> Stiction!/1
  Sign1/1 -> reverse/1
  sliding friction coefficient/1 -> Product/2
  Product/1 -> F_Slide [N]/1
  pos [m]/1 -> posFP [m]/1
  vel [m/s]/1 -> Abs/1, Sign1/1
  F_Normal [N]/1 -> sliding friction coefficient/1
  reverse/1 -> Product/1

== system rolling_contact_36_example/36-Point Sliding Contact Model/Body Contact 26/Ground Friction Model/X-Axis Static Friction Model ==
  note: Static Friction Model
  note: Stiction Limit Detector
  note: Zero multiplication prevents
      | horizontal friction model from
      | oscillating between static and kinetic
      | friction when the vertical force is zero but
      | the ground level is not yet reached
      | in the upward motion
  F_Normal [N] : Inport
  pos [m] : Inport  Port=2
  vel [m/s] : Inport  Port=3
  posFP [m] : Inport  Port=4
  Enable : EnablePort  StatesWhenEnabling=reset  ZeroCross=off
  Abs : Abs  SaturateOnIntegerOverflow=off
  Abs. : Abs  SaturateOnIntegerOverflow=off
  Check Vertical Friction : Product  RndMeth=Zero
  FixPt Relational Operator : RelationalOperator  Operator=>  OutDataTypeStr=boolean  ZeroCross=off  InputSameDT=off
  Gain3 : Gain  Gain=k_gx
  Gain4 : Gain  Gain=1/v_gx_max
  Memory : Memory
  Mux1 : Mux  Inputs=2
  Positive : simulink/Logic and Bit Operations/Compare To Zero  relop=>  OutDataTypeStr=boolean
  Positive1 : simulink/Logic and Bit Operations/Compare To Zero  relop=>  OutDataTypeStr=boolean
  Sum : Sum  Inputs=-+
  Sum2 : Sum  Inputs=-+|
  X-Axis Stiction Force : Fcn  Expr=-u(1) * (1+sgn(u(1))*u(2))
  stiction limit force : Gain  Gain=mu_stick
  F_Stick [N] : Outport  OutputWhenDisabled=reset  InitialOutput=0
      settings: AttributesFormatString=when disabled: %<OutputWhenDisabled>\ninitial: %<InitialOutput>
  Sliding! : Outport  Port=2  OutputWhenDisabled=reset  InitialOutput=0
      settings: AttributesFormatString=when disabled: %<OutputWhenDisabled>\ninitial: %<InitialOutput>
  wires:
  F_Normal [N]/1 -> stiction limit force/1, Positive1/1
  Sum2/1 -> Gain3/1  "dx"
  pos [m]/1 -> Sum2/2
  posFP [m]/1 -> Sum2/1
  vel [m/s]/1 -> Gain4/1
  Sum/1 -> Positive/1
  Memory/1 -> FixPt Relational Operator/2
  Positive/1 -> FixPt Relational Operator/1, Memory/1
  Abs./1 -> Sum/2
  Mux1/1 -> X-Axis Stiction Force/1
  Gain3/1 -> Mux1/1
  Gain4/1 -> Mux1/2
  FixPt Relational Operator/1 -> Sliding!/1
  Abs/1 -> Sum/1
  stiction limit force/1 -> Abs/1
  X-Axis Stiction Force/1 -> Check Vertical Friction/1
  Positive1/1 -> Check Vertical Friction/2
  Check Vertical Friction/1 -> F_Stick [N]/1, Abs./1

== system rolling_contact_36_example/36-Point Sliding Contact Model/Body Contact 27/Ground Friction Model/Friction Switch ==
  note: Static/Kinetic Friction Switch
  Slide! : Inport
  Stick! : Inport  Port=2
  Memory : Memory
  S-R Flip-Flop : simulink_extras/Flip Flops/S-R Flip-Flop  initial_condition=1
  Terminator : Terminator
  Stiction : Outport
  wires:
  S-R Flip-Flop/1 -> Memory/1
  S-R Flip-Flop/2 -> Terminator/1
  Stick!/1 -> S-R Flip-Flop/1
  Slide!/1 -> S-R Flip-Flop/2
  Memory/1 -> Stiction/1

== system rolling_contact_36_example/36-Point Sliding Contact Model/Body Contact 27/Ground Friction Model/X-Axis Kinetic Friction Model ==
  note: Kinetic Friction Model
  note: Footpoint Determiner
  note: Sliding Limit Detector
  pos [m] : Inport
  vel [m/s] : Inport  Port=2
  F_Normal [N] : Inport  Port=3
  Enable : EnablePort  StatesWhenEnabling=reset  ZeroCross=off
  Abs : Abs  SaturateOnIntegerOverflow=off
  Constant : Constant  Value=vLimit
  FixPt Relational Operator : RelationalOperator  Operator=>  OutDataTypeStr=boolean  ZeroCross=off  InputSameDT=off
  Memory : Memory
  Negative : simulink/Logic and Bit Operations/Compare To Zero  relop=<  OutDataTypeStr=boolean
  Product : Product  RndMeth=Zero
  Sign1 : Signum
  Sum : Sum  Inputs=|+-
  reverse : Gain  Gain=-1
  sliding friction coefficient : Gain  Gain=mu_slide
  posFP [m] : Outport  InitialOutput=0
      settings: AttributesFormatString=initial = '%<InitialOutput>'\nwhen disabled = '%<OutputWhenDisabled>'
  Stiction! : Outport  Port=2  OutputWhenDisabled=reset  InitialOutput=0
      settings: AttributesFormatString=initial = '%<InitialOutput>'\nwhen disabled = '%<OutputWhenDisabled>'
  F_Slide [N] : Outport  Port=3  OutputWhenDisabled=reset  InitialOutput=0
      settings: AttributesFormatString=initial = '%<InitialOutput>'\nwhen disabled = '%<OutputWhenDisabled>'
  wires:
  reverse/1 -> Product/1
  F_Normal [N]/1 -> sliding friction coefficient/1
  vel [m/s]/1 -> Sign1/1, Abs/1
  pos [m]/1 -> posFP [m]/1
  Product/1 -> F_Slide [N]/1
  sliding friction coefficient/1 -> Product/2
  Sign1/1 -> reverse/1
  FixPt Relational Operator/1 -> Stiction!/1
  Memory/1 -> FixPt Relational Operator/2
  Negative/1 -> FixPt Relational Operator/1, Memory/1
  Abs/1 -> Sum/1
  Sum/1 -> Negative/1
  Constant/1 -> Sum/2
